simulink model "assignment"  (R2026a)
settings: Solver=ode45  StopTime=20  RelTol=1e-6
values from neighbouring files (symbols this model uses):
  A = [0 1 0 0; 0 -1 0 0; 0 0 0 1;0 1 g 0]    [assignment7_param.m]
  alpha = 1    [assignment7_param.m]
  B = [0; 1; 0; -1]    [assignment7_param.m]
  C = [1 0 0 0; 0 0 1 0]    [assignment7_param.m]
  Cs = [1 0 0 0]    [assignment7_param.m]
  K = place(A,-B,v)    [assignment7_param.m]
  L = Gamma - K * Pi    [assignment7_param.m]
  omega = 1    [assignment7_param.m]
  P = [0 0 0; 1 0 0; 0 0 0; -1 0 0]    [assignment7_param.m]
  Q = [0 -1 0]    [assignment7_param.m]
settings Model: Creator=luca-callegari  LastModifiedBy=saradenti

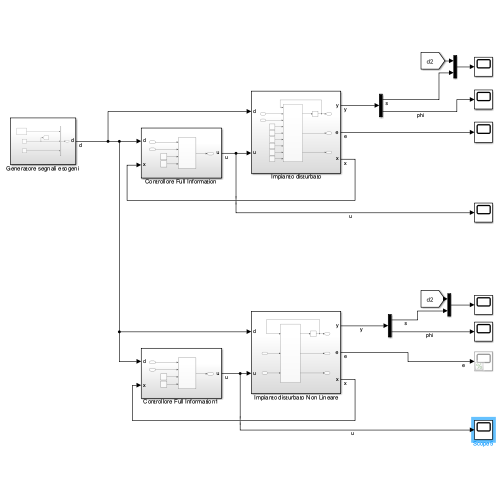
[thumbnail: Simulink's stored preview of the top-level diagram]
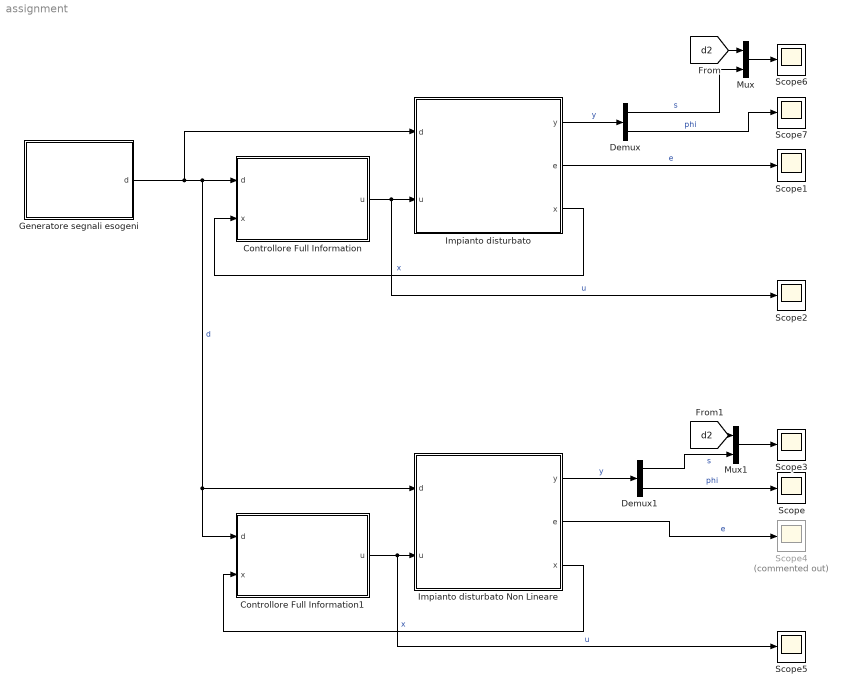
== system assignment ==
  " Impianto disturbato" : Subsystem
  " Impianto disturbato Non Lineare" : Subsystem
  Controllore Full Information : Subsystem
  Controllore Full Information1 : Subsystem
  Demux : Demux  Outputs=2
  Demux1 : Demux  Outputs=2
  Generatore segnali esogeni : Subsystem
  Mux : Mux  Inputs=2
  Mux1 : Mux  Inputs=2
  Scope{,1..3,5..7} (7 alike) : Scope
      Scope settings: ActiveDisplayYMinimum=-9.8464232724317835  ActiveDisplayYMaximum=8.9136553335807385  DataLoggingVariableName=ScopeData4
      Scope1 settings: ActiveDisplayYMinimum=-2.1136945762755057  ActiveDisplayYMaximum=8.0562232527272091
      Scope2 settings: ActiveDisplayYMinimum=-252.77408086035828  ActiveDisplayYMaximum=200.41348178202171  DataLoggingVariableName=ScopeData2
      Scope3 settings: DataLoggingVariableName=ScopeData7
      Scope5 settings: ActiveDisplayYMinimum=-2.6992239612993613E+11  ActiveDisplayYMaximum=2.4293015642622676E+12  DataLoggingVariableName=ScopeData6
      Scope6 settings: ActiveDisplayYMinimum=-1  ActiveDisplayYMaximum=1
      Scope7 settings: ActiveDisplayYMinimum=0.79352174687867683  ActiveDisplayYMaximum=0.81113757511672269  DataLoggingVariableName=ScopeData3
  Scope4 : Scope  Commented=on
      settings: ActiveDisplayYMinimum=-8.5981584018192764E+10  ActiveDisplayYMaximum=7.7383425615275513E+11  DataLoggingVariableName=ScopeData5
  wires:
  Controllore Full Information/1(u) -> Scope2/1, " Impianto disturbato"/2(u)  "u"
  " Impianto disturbato"/3(x) -> Controllore Full Information/2(x)  "x"
  " Impianto disturbato"/1(y) -> Demux/1  "y"
  Demux/2 -> Scope7/1  "phi"
  Generatore segnali esogeni/1(d) -> " Impianto disturbato"/1(d), " Impianto disturbato Non Lineare"/1(d), Controllore Full Information1/1(d), Controllore Full Information/1(d)  "d"
  " Impianto disturbato Non Lineare"/3(x) -> Controllore Full Information1/2(x)  "x"
  " Impianto disturbato"/2(e) -> Scope1/1  "e"
  Controllore Full Information1/1(u) -> Scope5/1, " Impianto disturbato Non Lineare"/2(u)  "u"
  " Impianto disturbato Non Lineare"/1(y) -> Demux1/1  "y"
  " Impianto disturbato Non Lineare"/2(e) -> Scope4/1  "e"
  Demux1/1 -> Mux1/2  "s"
  Demux1/2 -> Scope/1  "phi"
  Mux/1 -> Scope6/1
  Demux/1 -> Mux/2  "s"
  [d2] -> Mux/1
  Mux1/1 -> Scope3/1
  [d2] -> Mux1/1

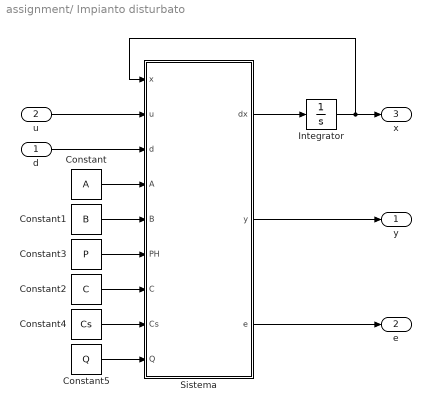
== system assignment/ Impianto disturbato ==
  d : Inport
  u : Inport  Port=2
  Constant : Constant  Value=A  VectorParams1D=off
  Constant1 : Constant  Value=B  VectorParams1D=off
  Constant2 : Constant  Value=C  VectorParams1D=off
  Constant3 : Constant  Value=P  VectorParams1D=off
  Constant4 : Constant  Value=Cs  VectorParams1D=off
  Constant5 : Constant  Value=Q  VectorParams1D=off
  Integrator : Integrator  InitialCondition=[0;0;0;0]
  Sistema : MATLAB Function  TreatAsAtomicUnit=on
  y : Outport
  e : Outport  Port=2
  x : Outport  Port=3
  wires:
  Sistema/1(dx) -> Integrator/1
  Integrator/1 -> Sistema/1(x), x/1
  Sistema/2(y) -> y/1
  u/1 -> Sistema/2(u)
  Constant/1 -> Sistema/4(A)
  Constant1/1 -> Sistema/5(B)
  Constant2/1 -> Sistema/7(C)
  d/1 -> Sistema/3(d)
  Constant3/1 -> Sistema/6(PH)
  Sistema/3(e) -> e/1
  Constant4/1 -> Sistema/8(Cs)
  Constant5/1 -> Sistema/9(Q)

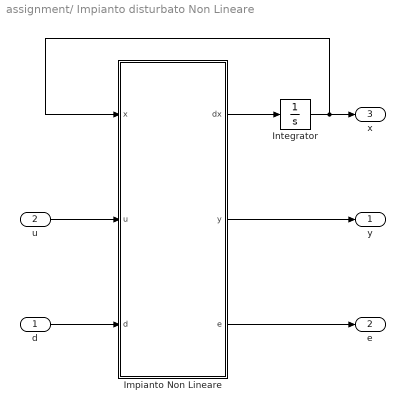
== system assignment/ Impianto disturbato Non Lineare ==
  d : Inport
  u : Inport  Port=2
  Impianto Non Lineare : MATLAB Function  TreatAsAtomicUnit=on
  Integrator : Integrator  InitialCondition=[0;0;0;0]
  y : Outport
  e : Outport  Port=2
  x : Outport  Port=3
  wires:
  Impianto Non Lineare/1(dx) -> Integrator/1
  Integrator/1 -> Impianto Non Lineare/1(x), x/1
  Impianto Non Lineare/2(y) -> y/1
  u/1 -> Impianto Non Lineare/2(u)
  d/1 -> Impianto Non Lineare/3(d)
  Impianto Non Lineare/3(e) -> e/1

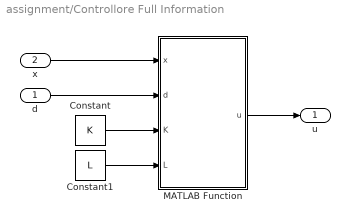
== system assignment/Controllore Full Information ==
  d : Inport
  x : Inport  Port=2
  Constant : Constant  Value=K  VectorParams1D=off
  Constant1 : Constant  Value=L  VectorParams1D=off
  MATLAB Function : MATLAB Function  TreatAsAtomicUnit=on
  u : Outport
  wires:
  MATLAB Function/1(u) -> u/1
  x/1 -> MATLAB Function/1(x)
  d/1 -> MATLAB Function/2(d)
  Constant/1 -> MATLAB Function/3(K)
  Constant1/1 -> MATLAB Function/4(L)

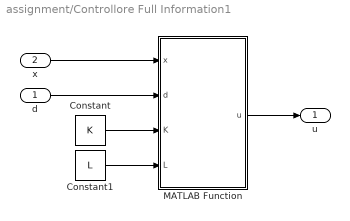
== system assignment/Controllore Full Information1 ==
  d : Inport
  x : Inport  Port=2
  Constant : Constant  Value=K  VectorParams1D=off
  Constant1 : Constant  Value=L  VectorParams1D=off
  MATLAB Function : MATLAB Function  TreatAsAtomicUnit=on
  u : Outport
  wires:
  MATLAB Function/1(u) -> u/1
  x/1 -> MATLAB Function/1(x)
  d/1 -> MATLAB Function/2(d)
  Constant/1 -> MATLAB Function/3(K)
  Constant1/1 -> MATLAB Function/4(L)

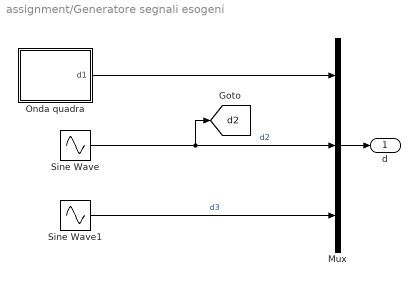
== system assignment/Generatore segnali esogeni ==
  Mux : Mux  Inputs=3
  Onda quadra : Subsystem
  Sine Wave : Sin  Amplitude=alpha  Frequency=omega  SampleTime=0
  Sine Wave1 : Sin  Amplitude=alpha*omega  Frequency=omega  Phase=pi/2  SampleTime=0
  d : Outport
  tag scope: d2=global
  wires:
  Sine Wave/1 -> Mux/2, [d2]  "d2"
  Sine Wave1/1 -> Mux/3  "d3"
  Mux/1 -> d/1
  Onda quadra/1(d1) -> Mux/1

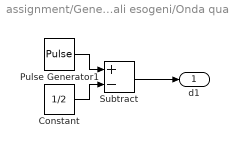
== system assignment/Generatore segnali esogeni/Onda quadra ==
  Constant : Constant  Value=1/2
  Pulse Generator1 : DiscretePulseGenerator  PulseType=Time based  Period=50  PulseWidth=50
  Subtract : Sum  Inputs=+-
  d1 : Outport
  wires:
  Constant/1 -> Subtract/2
  Pulse Generator1/1 -> Subtract/1
  Subtract/1 -> d1/1

== matlab function assignment/ Impianto disturbato/Sistema ==
  data: x input; dx output; u input; d input; y output; A input; B input; PH input; C input; Cs input; Q input; e output
function [dx, y, e] = fcn(x,u,d,A,B,PH,C,Cs,Q)
    dx = A*x + B*u + PH*d;
    y = C*x;
    e = Cs*x + Q*d;
end

== matlab function assignment/Controllore Full Information/MATLAB Function ==
  data: x input; d input; K input; u output; L input
function u = fcn(x,d,K,L)
    u = K*x + L*d;
end

== matlab function assignment/ Impianto disturbato Non Lineare/Impianto Non Lineare ==
  data: x input; dx output; u input; d input; y output; e output
function [dx, y, e] = fcn(x,u,d)
    dx = zeros(4,1);
    dx(1) = x(2);
    dx(2) = -x(2) + u + d(1);
    dx(3) = x(4);
    dx(4) = 9.81*sin(x(3)) - dx(2)*cos(x(3));
    
    y = zeros(2,1);
    y(1) = x(1);
    y(2) = x(3);

    e = x(1) - d(2);
end

== matlab function assignment/Controllore Full Information1/MATLAB Function ==
  data: x input; d input; K input; u output; L input
function u = fcn(x,d,K,L)
    u = K*x + L*d;
end
